simulink model "FCSMPC_double_vector_2025b"  (R2025b)
settings: Solver=FixedStepDiscrete  StartTime=0.0  StopTime=2  FixedStep=SimulinkTs  RelTol=1e-3
PreLoadFcn:
  | % Verzeichnis des Modells zum MATLAB-Pfad hinzufügen
  | modelDir = fileparts(get_param(bdroot, 'FileName'));
  | addpath(modelDir);
  | 
  | % Nur der Dateiname – kein Pfad!
  | set_param(bdroot, 'DataDictionary', 'FOC_params.sldd');
model workspace (MAT data in the model file):
  Np : Simulink.Parameter (value not decoded)
values from neighbouring files (symbols this model uses):
  Filter_Current_FilterTimeConst = 3.3333333333333335E-5    [FOC_params.sldd]
  Filter_Current_SensorTimeConst = 1.5915494309189535E-6    [FOC_params.sldd]
  FOC = evalin("base", "FOC")    [createFOC_SLDD.m]
  FOC_Control_Current_KIid = 10.0    [FOC_params.sldd]
  FOC_Control_Current_KIiq = 10.0    [FOC_params.sldd]
  FOC_Control_Current_KPid = 0.20418507462686566    [FOC_params.sldd]
  FOC_Control_Current_KPiq = 0.58674626865671642    [FOC_params.sldd]
  FOC_Control_Current_Krd = 0.8    [FOC_params.sldd]
  FOC_Control_Current_Krq = 0.8    [FOC_params.sldd]
  FOC_Control_Current_TclCur = 0.1    [FOC_params.sldd]
  FOC_Control_Current_Tnd = 0.1    [FOC_params.sldd]
  FOC_Control_Current_Tnq = 0.1    [FOC_params.sldd]
  FOC_Control_InverterVdc_V = 400.0    [FOC_params.sldd]
  FOC_Control_MotorImax_A = 650.0    [FOC_params.sldd]
  FOC_Control_MTPA_MTPV_nT_id_grid = -450.06704889786266 -439.56177000270145 -427.77784873303676 -416.66404703197372 -406.07553272717422 -395.15516533678584 -384.31176061747851 -374.03652088128132 -363.90551910193739 -353.79478643334204 -344.0221683092833 -334.51243453441936 -324.94614350292119 -315.21793409137081 -305.26543360965195 -295.21828280911944 -285.133916324101 -275.01232812136521 -264.86951532374729 -254.7797625148454 -244    [FOC_params.sldd]
  FOC_Control_MTPA_MTPV_nT_iq_grid = -449.09165648258488 -442.56958748923387 -437.25247759546528 -430.91792082419158 -423.83735797306491 -417.11730433547 -410.54064621830616 -403.71584331167304 -396.93611069310379 -390.15794305727007 -382.97216593027133 -375.44639668848538 -367.93447385667577 -360.57088856352266 -353.41289778449368 -346.34020584402072 -339.28416684923008 -332.22010880540631 -325.11927997033376 -317.92299905654966 -31    [FOC_params.sldd]
  FOC_Control_MTPA_MTPV_T_vec = -245.0 -240.0 -235.0 -230.0 -225.0 -220.0 -215.0 -210.0 -205.0 -200.0 -195.0 -190.0 -185.0 -180.0 -175.0 -170.0 -165.0 -160.0 -155.0 -150.0 -145.0 -140.0 -135.0 -130.0 -125.0 -120.0 -115.0 -110.0 -105.0 -100.0 -95.0 -90.0 -85.0 -80.0 -75.0 -70.0 -65.0 -60.0 -55.0 -50.0 -45.0 -40.0 -35.0 -30.0 -25.0 -20.0 -15.0 -10.0 -5.0 0.0 5.0 10.0 15.0 20.0 25.0 30.0 35.0 40.0 45.0 50.0 55.0 60.0 65.0 70.0 75.0    [FOC_params.sldd]
  FOC_Control_MTPA_MTPV_w_vec = 0.0 10.471975511965978 20.943951023931955 31.415926535897931 41.887902047863911 52.359877559829883 62.831853071795862 73.303828583761828 83.775804095727821 94.247779607693786 104.71975511965977 115.19173063162575 125.66370614359172 136.1356816555577 146.60765716752366 157.07963267948966 167.55160819145564 178.02358370342159 188.49555921538757 198.96753472735358 209.43951023931953 219.9114857512855    [FOC_params.sldd]
  FOC_Control_OpenLoop_Id_Ref_A = 0.0    [FOC_params.sldd]
  FOC_Control_OpenLoop_Iq_Ref_A = 0.0    [FOC_params.sldd]
  FOC_Control_OpenLoop_Ud_OpenLoop_V = 0.0    [FOC_params.sldd]
  FOC_Control_OpenLoop_Uq_OpenLoop_V = 0.0    [FOC_params.sldd]
  FOC_Control_RF_omegamech_rad_s = 3141.5926535897934    [FOC_params.sldd]
  FOC_Control_RF_RateCurrent_A = 500.0    [FOC_params.sldd]
  FOC_Control_RF_RateTrq_Nm = 500.0    [FOC_params.sldd]
  FOC_Control_theta_mechOffsetFix = 0.0    [FOC_params.sldd]
  FOC_Control_theta_mechOffsetTime = 0.0    [FOC_params.sldd]
  FOC_Control_TorqueRef_Nm = 10.0    [FOC_params.sldd]
  FOC_Control_Umax_V = 230.94010767585033    [FOC_params.sldd]
  FOC_Flag_ClosedLoopControl = 1.0    [FOC_params.sldd]
  FOC_Flag_ControlStrategy = 2.0    [FOC_params.sldd]
  FOC_Flag_PWMEnable = 1.0    [FOC_params.sldd]
  FOC_Flag_ResetControl = 0.0    [FOC_params.sldd]
  FOC_Flag_TorqueControl = 1.0    [FOC_params.sldd]
  FOC_LUT_DQLimiter_DQ_LUTScaling = 1.8749999999999995E-5    [FOC_params.sldd]
  FOC_PWM_AZSPWMMethod = 3.0    [FOC_params.sldd]
  FOC_PWM_HybridMode = 1.0    [FOC_params.sldd]
  FOC_PWM_LB1 = 0.5    [FOC_params.sldd]
  FOC_PWM_LB2 = 0.77    [FOC_params.sldd]
  FOC_PWM_PWMManuel = 1.0    [FOC_params.sldd]
  FOC_PWM_RSPWMMethod = 2.0    [FOC_params.sldd]
  FOC_PWM_UB1 = 0.66    [FOC_params.sldd]
  FOC_PWM_UB2 = 0.9    [FOC_params.sldd]
  FOC_SampleTime_TsCur = 0.0001    [FOC_params.sldd]
undefined symbols (not defined in the file or in its folder): dspblkCoreblockFVToolHelper, FCS, Filter, gcbh, Plant, SimulinkTs
libraries: hdlsllib x2, simulink x2, autolibfluxpmsm x1
(part 7 of 8)

== matlab function FCSMPC_double_vector_2025b/FCS_MPC/BuildModel/BuildModel/Discretize_PMSM1 ==
  data: Bd output size=[2 2]; Ld input; Ad output size=[2 2]; Lq input; Rs input; Psi input; wel input; fd output size=[2 1]; Ts input
function [Bd, Ad, fd] = Discretize_PMSM(Ld, Lq, Rs, Psi, wel, Ts)

Ac = [ -Rs/Ld,        wel*Lq/Ld;
    -wel*Ld/Lq,  -Rs/Lq ];

Bc = [ 1/Ld, 0;
    0,    1/Lq ];

fc = [ 0;
    -wel*Psi/Lq ];

% Augmented matrix: states (2) + voltage inputs (2) + affine (1) = 5
M = [ Ac, Bc, fc;
    zeros(3,5) ];

Md = expm(M * Ts);

Ad   = Md(1:2, 1:2);
Bd = Md(1:2, 3:4);     % maps v_dq -> state increment
fd   = Md(1:2, 5);     % back-EMF contribution per step

== matlab function FCSMPC_double_vector_2025b/FCS_MPC/BuildModel/BuildModel/Build_Model1 ==
  data: Ad input; fd input; Gamma output size=[2*Np 2]; Phi output size=[2*Np 1]; Lambdafsw_Ssquare output size=[3*Np 3*Np]; Lambdafsw_SE output size=[3*Np 3]; Apow output size=[2*(Np+1) 2]; Bs_TI output size=[2 3]; Vdc input; lambda_fsw input
function [Gamma, Phi, Lambdafsw_Ssquare, Lambdafsw_SE, Apow, Bs_TI]    = BuildModel(Ad, fd, Vdc, lambda_fsw)
Np = 5;
nu = 3;  ny = 2;
C  = eye(ny);
Apow = zeros(ny*(Np+1), ny);
Apow(1:ny, :) = eye(ny);
for m = 1:Np
    Apow(m*ny + (1:ny), :) = Apow((m-1)*ny + (1:ny), :) * Ad;
end
Bs_TI = switch_to_alphabeta(Vdc);

Gamma = zeros(ny*Np, ny);
Phi   = zeros(ny*Np, 1);
for i = 1:Np
    ri = (i-1)*ny + (1:ny);
    Gamma(ri,:) = C * Apow(i*ny + (1:ny), :);
    acc = zeros(ny,1);
    for m = 0:i-1, acc = acc + Apow(m*ny + (1:ny), :)*fd; end
    Phi(ri) = C * acc;
end

S = eye(nu*Np);
for i = 2:Np
    ri = (i-1)*nu + (1:nu);
    rj = (i-2)*nu + (1:nu);
    S(ri,rj) = -eye(nu);
end
E = [eye(nu); zeros(nu*(Np-1), nu)];
lambda_eff = max(lambda_fsw, 1e-6);
Lambdafsw_SE = lambda_eff * (S.'*E);
Lambdafsw_Ssquare =  lambda_eff*(S.'*S);


end

function Bs_TI = switch_to_alphabeta(Vdc)
Msw = eye(3) - ones(3)/3;
Tc  = (2/3) * [ 1, -1/2,      -1/2;
    0,  sqrt(3)/2, -sqrt(3)/2 ];   % Clarke (2x3)

Bs_TI = Tc * Vdc * Msw;                % 2x3

end

== matlab function FCSMPC_double_vector_2025b/FCS_MPC/SDA_Solve/SDA Solve/QP_Runtime_40k_Simplified_Hybrid ==
  data: H_exp input double size=[15 15]; H_emb input; U_unc_exp output double size=[15 1]; U_unc_emb output; Gamma input double size=[10 2]; Phi input double size=[10 1]; Lambdafsw_SE input double size=[15 3]; Upsil input double size=[10 15]; Bd input double size=[2 2]; Bs_TI input double size=[2 3]; deltaIdqBaseOffset input double size=[2 1]; deltaIdqState input double size=[2 2]; magnitudeGain input double size=[1 1]; phaseCompensation input double size=[2 2]; rippleAttenuation input double size=[1 1]; rippleDelay input double size=[1 1]; Sin_Cos_Theta input double size=[2 1]; idiqFiltered input double size=[2 1]; idiq_ref input double size=[2 1]; lambdaZeroEmbedded input; Ts input double size=[1 1]; U_applied input double size=[6 1]; controllerDelay input double size=[1 1]; iabcPredictedPrevious input double size=[3 1]; Iabc_Motor input double size=[3 1]; predictionValid input boolean size=[1 1]; iabcReconstruction output double size=[3 1]; deltaIabcBase output double size=[3 1]; deltaIabcSwitch output double size=[3 3]; predictionError output double size=[3 1]; reconstructionError output double size=[3 1]; predictionError_dq output double size=[2 1]; reconstructionError_dq output double size=[2 1]; iabcAverageEstimated output double size=[3 1]; iabcRippleEstimated output double size=[3 1]; rippleResidual output double size=[3 1]; iabcSwitchCorrectionRaw output double size=[3 1]
function [U_unc_exp,U_unc_emb,iabcReconstruction, ...
    deltaIabcBase,deltaIabcSwitch, ...
    predictionError,reconstructionError, ...
    predictionError_dq,reconstructionError_dq, ...
    iabcAverageEstimated,iabcRippleEstimated,rippleResidual, ...
    iabcSwitchCorrectionRaw] = ...
    QP_Runtime_40k_Simplified_Hybrid( ...
    H_exp,H_emb,Gamma,Phi,Lambdafsw_SE,Upsil,Bd,Bs_TI, ...
    deltaIdqBaseOffset,deltaIdqState,magnitudeGain,phaseCompensation, ...
    rippleAttenuation,rippleDelay,Sin_Cos_Theta,idiqFiltered, ...
    idiq_ref,lambdaZeroEmbedded,Ts,U_applied,controllerDelay, ...
    iabcPredictedPrevious,Iabc_Motor,predictionValid)
%#codegen
%QP_RUNTIME_40K_SIMPLIFIED_HYBRID Standalone hybrid runtime calculation.
% Current reconstruction is evaluated once. The two matched unconstrained
% centers are then formed using their respective factors and linear terms.

Ts = max(realmin('double'),double(Ts));
idiqFiltered = double(idiqFiltered); idiq_ref = double(idiq_ref);
U_applied = double(U_applied);
lambdaZeroEmbedded = max(0.0,double(lambdaZeroEmbedded));
Bd = double(Bd); Bs_TI = double(Bs_TI);
Sin_Cos_Theta = double(Sin_Cos_Theta);
iabcPredictedPrevious = double(iabcPredictedPrevious);
Iabc_Motor = double(Iabc_Motor);
predictionValid = logical(predictionValid);
uFirst = U_applied(1:3); uSecond = U_applied(4:6);
uAverage = 0.5*(uFirst+uSecond);

sinTheta = Sin_Cos_Theta(1); cosTheta = Sin_Cos_Theta(2);
Rp = [cosTheta, sinTheta; -sinTheta, cosTheta];
TinvClarke = [1.0, 0.0; -0.5, sqrt(3)/2; -0.5, -sqrt(3)/2];
Tclarke = [2/3, -1/3, -1/3; 0, 1/sqrt(3), -1/sqrt(3)];
Tdq2abc = TinvClarke*Rp.'; Tabc2dq = Rp*Tclarke;
deltaIdqSwitch = Bd*Rp*Bs_TI;

deltaIdqBase = deltaIdqState*idiqFiltered+deltaIdqBaseOffset;
period = 2.0*Ts;
rippleAtMeasurementDq = ripple_at_phase( ...
    deltaIdqSwitch,uFirst,uSecond,uAverage,Ts,period-rippleDelay);
rippleResidualDq = ...
    magnitudeGain*rippleAttenuation*rippleAtMeasurementDq;
idiqAverage = phaseCompensation*( ...
    magnitudeGain*idiqFiltered-rippleResidualDq);
idiqAverage = idiqAverage+(rippleDelay/Ts)*( ...
    deltaIdqBase+deltaIdqSwitch*uAverage);
rippleNow = ripple_at_phase( ...
    deltaIdqSwitch,uFirst,uSecond,uAverage,Ts,period);
idiqAtSample = idiqAverage+rippleNow;
delayRatio = min(max(0.0,double(controllerDelay)),Ts)/Ts;
idiqCompensated = idiqAtSample+delayRatio*( ...
    deltaIdqBase+deltaIdqSwitch*uSecond);

iabcReconstruction = Tdq2abc*idiqCompensated;
deltaIabcBase = Tdq2abc*deltaIdqBase;
deltaIabcSwitch = Tdq2abc*deltaIdqSwitch;
iabcAverageEstimated = Tdq2abc*idiqAverage;
iabcRippleEstimated = Tdq2abc*rippleNow;
rippleResidual = Tdq2abc*rippleResidualDq;
iabcAmpCorrected = Tdq2abc*(magnitudeGain*idiqFiltered);
iabcSwitchCorrectionRaw = ...
    (iabcAverageEstimated-iabcAmpCorrected)+iabcRippleEstimated;
if predictionValid
    predictionError = iabcReconstruction-iabcPredictedPrevious;
else
    predictionError = zeros(3,1);
end
reconstructionError = Iabc_Motor-iabcReconstruction;
predictionError_dq = Tabc2dq*predictionError;
reconstructionError_dq = Tabc2dq*reconstructionError;

Np = 5;
r = Gamma*idiqCompensated+Phi-repmat(idiq_ref,Np,1);
F_exp = Upsil.'*r-Lambdafsw_SE*uSecond;
FzeroEmbedded = -0.75*lambdaZeroEmbedded*ones(3*Np,1);
F_emb = F_exp+FzeroEmbedded;
y_exp = H_exp.'\(-F_exp);
U_unc_exp = H_exp\y_exp;
y_emb = H_emb.'\(-F_emb);
U_unc_emb = H_emb\y_emb;
end

function rippleCurrent = ripple_at_phase( ...
    deltaSwitch,uFirst,uSecond,uAverage,vectorStep,t)
period = 2.0*vectorStep;
deltaFirst = deltaSwitch*(uFirst-uAverage);
deltaSecond = deltaSwitch*(uSecond-uAverage);
rippleStart = -0.5*deltaFirst;
t = min(max(0.0,t),period);
if t <= vectorStep
    rippleCurrent = rippleStart+(t/vectorStep)*deltaFirst;
else
    rippleCurrent = rippleStart+deltaFirst+ ...
        ((t-vectorStep)/vectorStep)*deltaSecond;
end
end

== matlab function FCSMPC_double_vector_2025b/FCS_MPC/SDA_Solve/SDA Solve/ SDA_Solve_Synchronized1 ==
  data: H_exp input double size=[15 15]; Jopt output double size=[1 1]; U_unc_exp input double size=[15 1]; H_emb input; U_unc_emb input; NmaxNod input double size=[1 1]; UoptPrev input double size=[15 1]; iabcCompensated input double size=[3 1]; deltaIabcBase input double size=[3 1]; deltaIabcSwitch input double size=[3 3]; lambdaZero input double size=[1 1]; lambdaDeadtime input double size=[1 1]; deadtime_ratio input double size=[1 1]; currentEpsMargin input double size=[1 1]; nodes output double size=[1 1]; optimal output boolean size=[1 1]; Uopt output double size=[15 1]; Uapply output double size=[6 1]; predictionValidNext output boolean size=[1 1]; iabcPredictedNext output double size=[3 1]; leafNodes output double size=[1 1]; bestCMVCost output double size=[1 1]; cmvMetricRatio output double size=[1 1]; switchCountApplied output double size=[1 1]; debug_lower output double size=[3 1]; debug_upper output double size=[3 1]; Jround output double size=[1 1]; Jshift output double size=[1 1]; JbabaiEmbedded output; JbabaiExplicit output; initialRadius output; solutionToggle output boolean size=[1 1]
function [Jopt, nodes, optimal, Uopt, Uapply, ...
    predictionValidNext,iabcPredictedNext, ...
    leafNodes, bestCMVCost, cmvMetricRatio, switchCountApplied, ...
    debug_lower, debug_upper, Jround, Jshift, ...
    JbabaiEmbedded, JbabaiExplicit, initialRadius, solutionToggle] = ...
    SDA_Solve_Synchronized_Hybrid( ...
    H_exp, U_unc_exp, H_emb, U_unc_emb, NmaxNod, UoptPrev, ...
    iabcCompensated, deltaIabcBase, deltaIabcSwitch, ...
    lambdaZero, lambdaDeadtime, deadtime_ratio, currentEpsMargin)
%#codegen
%SDA_SOLVE_SYNCHRONIZED_HYBRID Embedded Babai plus explicit SDA search.
% H_emb/U_unc_emb determine one Babai candidate. That binary sequence is
% re-evaluated under the explicit objective and becomes the initial
% incumbent. Every tree-search center, residual and branch penalty then
% uses H_exp/U_unc_exp. Feed Uopt back through the existing Unit Delay.

Np = 5;
nu = 3;
n = numel(U_unc_exp);

UbarExp = H_exp*U_unc_exp;
UbarEmb = H_emb*U_unc_emb;
uprev = UoptPrev(4:6);
deadtimeRatio = deadtime_ratio;

Uround = min(max(round(U_unc_exp),0.0),1.0);
Ushift = zeros(n,1);
Ushift(1:n-nu) = UoptPrev(nu+1:n);
Ushift(n-nu+1:n) = UoptPrev(n-nu+1:n);

% Forward Babai nearest-plane point for the embedded factor.
% This uses the same conditional centers and binary tie rule as the first
% Schnorr--Euchner descent, but constructs a complete incumbent without
% backtracking.
Ubabai = zeros(n,1);
for babaiLevel = 1:n
    babaiHead = 0.0;
    if babaiLevel > 1
        babaiHead = H_emb(babaiLevel,1:babaiLevel-1)* ...
            Ubabai(1:babaiLevel-1);
    end
    babaiCenter = (UbarEmb(babaiLevel)-babaiHead)/ ...
        H_emb(babaiLevel,babaiLevel);
    if babaiCenter <= 0.5
        Ubabai(babaiLevel) = 0.0;
    else
        Ubabai(babaiLevel) = 1.0;
    end
end

Jround = norm(H_exp*(Uround-U_unc_exp),2)^2;
Jshift = norm(H_exp*(Ushift-U_unc_exp),2)^2;
JbabaiEmbedded = norm(H_emb*(Ubabai-U_unc_emb),2)^2;
JbabaiExplicit = norm(H_exp*(Ubabai-U_unc_exp),2)^2;

% The embedded Babai sequence is the hybrid initializer. Re-evaluating it
% with the explicit factor avoids relying on a hard-coded constant offset.
Uini = Ubabai;
Jini = JbabaiExplicit;

bestCMVCost = sequence_cmv_cost_predicted( ...
    Uini,uprev,iabcCompensated,Np,nu, ...
    deltaIabcBase,deltaIabcSwitch,lambdaZero,lambdaDeadtime, ...
    deadtimeRatio,currentEpsMargin);
bestMetric = Jini+bestCMVCost;
initialRadius = bestMetric;
Uopt = Uini;

U = zeros(n,1);
kidx = ones(n,1);
d2s = zeros(n+1,1);
cmvD2s = zeros(n+1,1);
iabcPrediction = zeros(3,Np+1);
iabcPrediction(:,1) = iabcCompensated;
nodes = 0;
leafNodes = 0;
optimal = true;
i = 1;

while i >= 1
    if kidx(i) > 2
        kidx(i) = 1;
        i = i-1;
        continue;
    end
    head = 0.0;
    if i > 1
        head = H_exp(i,1:i-1)*U(1:i-1);
    end
    center = (UbarExp(i)-head)/H_exp(i,i);
    if center <= 0.5
        firstCandidate = 0.0;
    else
        firstCandidate = 1.0;
    end
    if kidx(i) == 1
        candidate = firstCandidate;
    else
        candidate = 1.0-firstCandidate;
    end
    kidx(i) = kidx(i)+1;
    U(i) = candidate;
    nodes = nodes+1;
    if NmaxNod > 0 && nodes > NmaxNod
        optimal = false;
        break;
    end

    residual = UbarExp(i)-head-H_exp(i,i)*candidate;
    metricNew = d2s(i)+residual*residual;
    cmvMetricNew = cmvD2s(i);
    if mod(i,nu) == 0
        predictionStep = i/nu;
        blockStart = i-nu+1;
        uCurrent = U(blockStart:i);
        if predictionStep == 1
            uPrevious = uprev;
        else
            uPrevious = U(blockStart-nu:blockStart-1);
        end
        iabcBeforeSwitch = iabcPrediction(:,predictionStep);
        [deltaStep,deltaDead] = deadtime_corrected_current_step( ...
            uPrevious,uCurrent,iabcBeforeSwitch, ...
            deltaIabcBase,deltaIabcSwitch,deadtimeRatio,currentEpsMargin);
        cmvIncrement = cmv_cost( ...
            uPrevious,uCurrent,iabcBeforeSwitch,deltaDead, ...
            lambdaZero,lambdaDeadtime,currentEpsMargin);
        metricNew = metricNew+cmvIncrement;
        cmvMetricNew = cmvMetricNew+cmvIncrement;
        iabcPrediction(:,predictionStep+1) = iabcBeforeSwitch+deltaStep;
    end
    if metricNew > bestMetric
        continue;
    end
    if i == n
        leafNodes = leafNodes+1;
        if metricNew < bestMetric
            bestMetric = metricNew;
            Uopt = U;
            bestCMVCost = cmvMetricNew;
        end
    else
        d2s(i+1) = metricNew;
        cmvD2s(i+1) = cmvMetricNew;
        i = i+1;
        kidx(i) = 1;
    end
end

if ~isfinite(bestMetric)
    Uopt = repmat(uprev,Np,1);
end

Uapply = Uopt(1:6);
UapplyFirst = Uopt(1:3);
UapplySecond = Uopt(4:6);

[deltaFirst,~] = deadtime_corrected_current_step( ...
    uprev,UapplyFirst,iabcCompensated, ...
    deltaIabcBase,deltaIabcSwitch, ...
    deadtimeRatio,currentEpsMargin);
iabcAfterFirst = iabcCompensated + deltaFirst;

[deltaSecond,~] = deadtime_corrected_current_step( ...
    UapplyFirst,UapplySecond,iabcAfterFirst, ...
    deltaIabcBase,deltaIabcSwitch,deadtimeRatio,currentEpsMargin);
iabcPredictedNext = iabcAfterFirst+deltaSecond;

switchCountApplied = sum(abs(UapplyFirst-uprev))+ ...
    sum(abs(UapplySecond-UapplyFirst));
Jopt = bestMetric;
if Jopt > eps
    cmvMetricRatio = bestCMVCost/Jopt;
else
    cmvMetricRatio = 0.0;
end
[~,debugDeltaDead] = deadtime_corrected_current_step( ...
    uprev,UapplyFirst,iabcCompensated,deltaIabcBase,deltaIabcSwitch, ...
    deadtimeRatio,currentEpsMargin);
[~,debug_lower,debug_upper] = cmv_cost( ...
    uprev,UapplyFirst,iabcCompensated,debugDeltaDead, ...
    lambdaZero,lambdaDeadtime,currentEpsMargin);
predictionValidNext = true;

% Toggle once after every completed SDA solution. The downstream switch
% detects this edge and explicitly restarts from the first vector.
persistent solutionToggleState
if isempty(solutionToggleState)
    solutionToggleState = false;
end
solutionToggleState = ~solutionToggleState;
solutionToggle = solutionToggleState;
end

function [deltaStep,deltaDead] = deadtime_corrected_current_step( ...
    uPrevious,uCurrent,iabcBeforeSwitch, ...
    deltaBase,deltaSwitch,deadtimeRatio,currentEps)
uDead = uCurrent;
changed = (uPrevious ~= uCurrent);
signEps = 0.1*currentEps;
for phase = 1:3
    if ~changed(phase)
        continue;
    end
    iPhase = iabcBeforeSwitch(phase);
    if iPhase >= signEps
        uDead(phase) = 0.0;
    elseif iPhase <= -signEps
        uDead(phase) = 1.0;
    else
        uDead(phase) = 0.5*(1.0-iPhase/signEps);
    end
end
uEffective = deadtimeRatio*uDead+(1.0-deadtimeRatio)*uCurrent;
deltaDead = deadtimeRatio*(deltaBase+deltaSwitch*uDead);
deltaStep = deltaBase+deltaSwitch*uEffective;
end

function [penalty,lowerBound,upperBound] = cmv_cost( ...
    uPrevious,uCurrent,iabcBeforeSwitch,deltaDead, ...
    lambdaZero,lambdaDeadtime,currentEpsMargin)
penalty = 0.0;
iabcDeadEnd = iabcBeforeSwitch+deltaDead;
lowerBound = min(iabcBeforeSwitch,iabcDeadEnd)-currentEpsMargin;
upperBound = max(iabcBeforeSwitch,iabcDeadEnd)+currentEpsMargin;
uncertain = (lowerBound <= 0.0) & (upperBound >= 0.0);
if all(uCurrent == 0.0) || all(uCurrent == 1.0)
    penalty = penalty+lambdaZero;
end
changed = (uPrevious ~= uCurrent);
if sum(changed) ~= 2
    return;
end
canBeZero = false(3,1);
canBeOne = false(3,1);
for phase = 1:3
    if ~changed(phase)
        canBeZero(phase) = (uPrevious(phase) == 0.0);
        canBeOne(phase) = (uPrevious(phase) == 1.0);
    elseif uncertain(phase)
        canBeZero(phase) = true;
        canBeOne(phase) = true;
    elseif iabcDeadEnd(phase) > 0.0
        canBeZero(phase) = true;
    else
        canBeOne(phase) = true;
    end
end
if all(canBeZero) || all(canBeOne)
    penalty = penalty+lambdaDeadtime;
end
end

function totalPenalty = sequence_cmv_cost_predicted( ...
    U,uprev,iabcInitial,Np,nu,deltaBase,deltaSwitch, ...
    lambdaZero,lambdaDeadtime,deadtimeRatio,currentEpsMargin)
totalPenalty = 0.0;
uPrevious = uprev;
iabcBeforeSwitch = iabcInitial;
for step = 1:Np
    rows = (step-1)*nu+(1:nu);
    uCurrent = U(rows);
    [deltaStep,deltaDead] = deadtime_corrected_current_step( ...
        uPrevious,uCurrent,iabcBeforeSwitch,deltaBase,deltaSwitch, ...
        deadtimeRatio,currentEpsMargin);
    totalPenalty = totalPenalty+cmv_cost( ...
        uPrevious,uCurrent,iabcBeforeSwitch,deltaDead, ...
        lambdaZero,lambdaDeadtime,currentEpsMargin);
    iabcBeforeSwitch = iabcBeforeSwitch+deltaStep;
    uPrevious = uCurrent;
end
end

== stateflow chart FCSMPC_double_vector_2025b/FCS_MPC/CurrentRefCalc/Current_RateLimiter/RateLimiter ==
  settings: updateMethod=DISCRETE  sampleTime=FOC.SampleTime.TsSpeed
  state IDLE
  state Rising
    entry:  y =  fi(y_prev +dT * R, 1, 32, 18);
    exit: y_prev = y;
  state Falling
    entry:  y = fi(y_prev+dT * F, 1, 32, 18);
    exit: y_prev = y;
  state Directpassage
    entry:  y = u;
    exit: y_prev = y;
  (default) -> IDLE
  IDLE -> (junction 22)
  (junction 22) -> Rising [order 1] : [(u-y_prev)/dT>=R]
  (junction 22) -> Falling [order 2] : [(u-y_prev)/dT<=F]
  Rising -> (junction 22)
  Falling -> (junction 22)
  Directpassage -> (junction 22)
  (junction 22) -> Directpassage [order 3] : [(u-y_prev)/dT<R && (u-y_prev)/dT>F]
  data: u input fixdt(1,32,18); R input fixdt(1,32,18); F input fixdt(1,32,18); dT constant fixdt(1,32,18) size=1 =FOC.SampleTime.TsSpeed; y output fixdt(1,32,18); y_prev local fixdt(1,32,18) =0

== matlab function FCSMPC_double_vector_2025b/FCS_MPC/SDA_Solve/SDA Solve/ SDA_Solve_Synchronized2 ==
  data: H_exp input double size=[15 15]; Jopt output double size=[1 1]; U_unc_exp input double size=[15 1]; H_emb input; U_unc_emb input; NmaxNod input double size=[1 1]; UoptPrev input double size=[15 1]; iabcCompensated input double size=[3 1]; deltaIabcBase input double size=[3 1]; deltaIabcSwitch input double size=[3 3]; lambdaZero input double size=[1 1]; lambdaDeadtime input double size=[1 1]; deadtime_ratio input double size=[1 1]; currentEpsMargin input double size=[1 1]; nodes output double size=[1 1]; optimal output boolean size=[1 1]; Uopt output double size=[15 1]; Uapply output double size=[6 1]; predictionValidNext output boolean size=[1 1]; iabcPredictedNext output double size=[3 1]; leafNodes output double size=[1 1]; bestCMVCost output double size=[1 1]; cmvMetricRatio output double size=[1 1]; switchCountApplied output double size=[1 1]; debug_lower output double size=[3 1]; debug_upper output double size=[3 1]; Jround output double size=[1 1]; Jshift output double size=[1 1]; JbabaiEmbedded output; JbabaiExplicit output; initialRadius output; solutionToggle output boolean size=[1 1]; currentLimit input; feasibleSolutionFound output; babaiPrefixFeasible output; prefixRepairUsed output; feasiblePrefixCount output; currentPruneCount output
function [Jopt, nodes, optimal, Uopt, Uapply, ...
    predictionValidNext,iabcPredictedNext, ...
    leafNodes, bestCMVCost, cmvMetricRatio, switchCountApplied, ...
    debug_lower, debug_upper, Jround, Jshift, ...
    JbabaiEmbedded, JbabaiExplicit, initialRadius, solutionToggle, ...
    feasibleSolutionFound, babaiPrefixFeasible, prefixRepairUsed, ...
    feasiblePrefixCount, currentPruneCount] = ...
    SDA_Solve_Synchronized_Hybrid_CurrentConstrained( ...
    H_exp, U_unc_exp, H_emb, U_unc_emb, NmaxNod, UoptPrev, ...
    iabcCompensated, deltaIabcBase, deltaIabcSwitch, ...
    lambdaZero, lambdaDeadtime, deadtime_ratio, currentEpsMargin, ...
    currentLimit)
%#codegen
%SDA_SOLVE_SYNCHRONIZED_HYBRID_CURRENTCONSTRAINED
% Current-constrained extension of SDA_Solve_Synchronized_Hybrid.
%
% The ordinary embedded Babai sequence remains the fast path. Its first two
% switching blocks, which are applied before the next controller transaction,
% are checked at both the dead-time endpoint and the vector endpoint. If that
% prefix is infeasible, all feasible two-block prefixes are scored only by the
% six-level embedded partial metric. The best prefix is completed once with a
% conditional embedded Babai suffix and reevaluated with the full explicit
% objective. The explicit search retains every feasible prefix and performs
% current pruning after each of the first two complete switching blocks.
%
% currentLimit is a phase-current peak limit in amperes. A nonpositive or
% nonfinite value disables the current constraint for diagnostic use.

Np = 5;
nu = 3;
n = numel(U_unc_exp);
constrainedBlocks = 2;

UbarExp = H_exp*U_unc_exp;
UbarEmb = H_emb*U_unc_emb;
uprev = UoptPrev(4:6);
deadtimeRatio = deadtime_ratio;
constraintEnabled = isfinite(currentLimit) && currentLimit > 0.0;

Uround = min(max(round(U_unc_exp),0.0),1.0);
Ushift = zeros(n,1);
Ushift(1:n-nu) = UoptPrev(nu+1:n);
Ushift(n-nu+1:n) = UoptPrev(n-nu+1:n);

% Ordinary embedded Babai candidate.
Ubabai = zeros(n,1);
for babaiLevel = 1:n
    babaiHead = 0.0;
    if babaiLevel > 1
        babaiHead = H_emb(babaiLevel,1:babaiLevel-1)* ...
            Ubabai(1:babaiLevel-1);
    end
    babaiCenter = (UbarEmb(babaiLevel)-babaiHead)/ ...
        H_emb(babaiLevel,babaiLevel);
    Ubabai(babaiLevel) = double(babaiCenter > 0.5);
end

Jround = norm(H_exp*(Uround-U_unc_exp),2)^2;
Jshift = norm(H_exp*(Ushift-U_unc_exp),2)^2;
JbabaiEmbedded = norm(H_emb*(Ubabai-U_unc_emb),2)^2;
JbabaiExplicit = norm(H_exp*(Ubabai-U_unc_exp),2)^2;

[babaiCMVCost,babaiPrefixFeasible] = evaluate_sequence( ...
    Ubabai,uprev,iabcCompensated,Np,nu, ...
    deltaIabcBase,deltaIabcSwitch,lambdaZero,lambdaDeadtime, ...
    deadtimeRatio,currentEpsMargin,currentLimit, ...
    constrainedBlocks,constraintEnabled);

prefixRepairUsed = false;
feasiblePrefixCount = 0;
hasFeasibleIncumbent = false;
Uini = zeros(n,1);
Jini = inf;
bestCMVCost = 0.0;

if babaiPrefixFeasible
    % Preserve the existing hybrid fast path exactly when it is feasible.
    Uini = Ubabai;
    Jini = JbabaiExplicit;
    bestCMVCost = babaiCMVCost;
    hasFeasibleIncumbent = true;
else
    prefixRepairUsed = true;
    bestPrefixMetric = inf;
    bestPrefix = zeros(2*nu,1);

    % Enumerate only the physical two-vector prefix. No Babai suffix is
    % formed inside this loop. The selected prefix is the feasible point
    % nearest to the unconstrained center in the first six embedded rows.
    for state1 = 0:7
        u1 = state_from_index(state1);
        [delta1,deltaDead1] = deadtime_corrected_current_step( ...
            uprev,u1,iabcCompensated,deltaIabcBase,deltaIabcSwitch, ...
            deadtimeRatio,currentEpsMargin);
        iDead1 = iabcCompensated+deltaDead1;
        iAfter1 = iabcCompensated+delta1;
        if ~current_is_feasible(iDead1,iAfter1,currentLimit, ...
                constraintEnabled)
            continue;
        end

        for state2 = 0:7
            u2 = state_from_index(state2);
            [delta2,deltaDead2] = deadtime_corrected_current_step( ...
                u1,u2,iAfter1,deltaIabcBase,deltaIabcSwitch, ...
                deadtimeRatio,currentEpsMargin);
            iDead2 = iAfter1+deltaDead2;
            iAfter2 = iAfter1+delta2;
            if ~current_is_feasible(iDead2,iAfter2,currentLimit, ...
                    constraintEnabled)
                continue;
            end

            feasiblePrefixCount = feasiblePrefixCount+1;
            prefix = [u1;u2];
            prefixResidual = UbarEmb(1:2*nu)- ...
                H_emb(1:2*nu,1:2*nu)*prefix;
            prefixMetric = prefixResidual.'*prefixResidual;
            if prefixMetric < bestPrefixMetric
                bestPrefixMetric = prefixMetric;
                bestPrefix = prefix;
            end
        end
    end

    if feasiblePrefixCount > 0
        % Compute exactly one conditional embedded Babai suffix.
        Uini(1:2*nu) = bestPrefix;
        for babaiLevel = 2*nu+1:n
            babaiHead = H_emb(babaiLevel,1:babaiLevel-1)* ...
                Uini(1:babaiLevel-1);
            babaiCenter = (UbarEmb(babaiLevel)-babaiHead)/ ...
                H_emb(babaiLevel,babaiLevel);
            Uini(babaiLevel) = double(babaiCenter > 0.5);
        end

        Jini = norm(H_exp*(Uini-U_unc_exp),2)^2;
        [bestCMVCost,initialCandidateFeasible] = evaluate_sequence( ...
            Uini,uprev,iabcCompensated,Np,nu, ...
            deltaIabcBase,deltaIabcSwitch,lambdaZero,lambdaDeadtime, ...
            deadtimeRatio,currentEpsMargin,currentLimit, ...
            constrainedBlocks,constraintEnabled);
        hasFeasibleIncumbent = initialCandidateFeasible;
    end
end

if hasFeasibleIncumbent
    bestMetric = Jini+bestCMVCost;
    Uopt = Uini;
else
    % An infeasible candidate may guide ordering but is never a finite upper
    % bound. The first feasible leaf found by the main search establishes it.
    bestMetric = inf;
    initialRadius = inf;
    Uopt = zeros(n,1);
    bestCMVCost = 0.0;
end
if hasFeasibleIncumbent
    initialRadius = bestMetric;
end

U = zeros(n,1);
kidx = ones(n,1);
d2s = zeros(n+1,1);
cmvD2s = zeros(n+1,1);
iabcPrediction = zeros(3,Np+1);
iabcPrediction(:,1) = iabcCompensated;
nodes = 0;
leafNodes = 0;
currentPruneCount = 0;
optimal = true;
i = 1;

while i >= 1
    if kidx(i) > 2
        kidx(i) = 1;
        i = i-1;
        continue;
    end
    head = 0.0;
    if i > 1
        head = H_exp(i,1:i-1)*U(1:i-1);
    end
    center = (UbarExp(i)-head)/H_exp(i,i);
    firstCandidate = double(center > 0.5);
    if kidx(i) == 1
        candidate = firstCandidate;
    else
        candidate = 1.0-firstCandidate;
    end
    kidx(i) = kidx(i)+1;
    U(i) = candidate;
    nodes = nodes+1;
    if NmaxNod > 0 && nodes > NmaxNod
        optimal = false;
        break;
    end

    residual = UbarExp(i)-head-H_exp(i,i)*candidate;
    metricNew = d2s(i)+residual*residual;
    cmvMetricNew = cmvD2s(i);
    currentFeasible = true;
    if mod(i,nu) == 0
        predictionStep = i/nu;
        blockStart = i-nu+1;
        uCurrent = U(blockStart:i);
        if predictionStep == 1
            uPrevious = uprev;
        else
            uPrevious = U(blockStart-nu:blockStart-1);
        end
        iabcBeforeSwitch = iabcPrediction(:,predictionStep);
        [deltaStep,deltaDead] = deadtime_corrected_current_step( ...
            uPrevious,uCurrent,iabcBeforeSwitch, ...
            deltaIabcBase,deltaIabcSwitch,deadtimeRatio,currentEpsMargin);
        iabcDeadEnd = iabcBeforeSwitch+deltaDead;
        iabcAfterStep = iabcBeforeSwitch+deltaStep;

        if predictionStep <= constrainedBlocks
            currentFeasible = current_is_feasible( ...
                iabcDeadEnd,iabcAfterStep,currentLimit,constraintEnabled);
        end
        if ~currentFeasible
            currentPruneCount = currentPruneCount+1;
            continue;
        end

        cmvIncrement = cmv_cost( ...
            uPrevious,uCurrent,iabcBeforeSwitch,deltaDead, ...
            lambdaZero,lambdaDeadtime,currentEpsMargin);
        metricNew = metricNew+cmvIncrement;
        cmvMetricNew = cmvMetricNew+cmvIncrement;
        iabcPrediction(:,predictionStep+1) = iabcAfterStep;
    end

    if hasFeasibleIncumbent && metricNew > bestMetric
        continue;
    end
    if i == n
        leafNodes = leafNodes+1;
        if ~hasFeasibleIncumbent || metricNew < bestMetric
            bestMetric = metricNew;
            Uopt = U;
            bestCMVCost = cmvMetricNew;
            hasFeasibleIncumbent = true;
        end
    else
        d2s(i+1) = metricNew;
        cmvD2s(i+1) = cmvMetricNew;
        i = i+1;
        kidx(i) = 1;
    end
end

feasibleSolutionFound = hasFeasibleIncumbent;
if ~feasibleSolutionFound
    % Keep the output deterministic but mark it invalid explicitly. The caller
    % must provide a separately validated safety fallback for this condition.
    Uopt = repmat(uprev,Np,1);
    bestMetric = inf;
    bestCMVCost = 0.0;
end

Uapply = Uopt(1:6);
UapplyFirst = Uopt(1:3);
UapplySecond = Uopt(4:6);

[deltaFirst,~] = deadtime_corrected_current_step( ...
    uprev,UapplyFirst,iabcCompensated, ...
    deltaIabcBase,deltaIabcSwitch,deadtimeRatio,currentEpsMargin);
iabcAfterFirst = iabcCompensated+deltaFirst;
[deltaSecond,~] = deadtime_corrected_current_step( ...
    UapplyFirst,UapplySecond,iabcAfterFirst, ...
    deltaIabcBase,deltaIabcSwitch,deadtimeRatio,currentEpsMargin);
iabcPredictedNext = iabcAfterFirst+deltaSecond;

switchCountApplied = sum(abs(UapplyFirst-uprev))+ ...
    sum(abs(UapplySecond-UapplyFirst));
Jopt = bestMetric;
if isfinite(Jopt) && Jopt > eps
    cmvMetricRatio = bestCMVCost/Jopt;
else
    cmvMetricRatio = 0.0;
end
[~,debugDeltaDead] = deadtime_corrected_current_step( ...
    uprev,UapplyFirst,iabcCompensated,deltaIabcBase,deltaIabcSwitch, ...
    deadtimeRatio,currentEpsMargin);
[~,debug_lower,debug_upper] = cmv_cost( ...
    uprev,UapplyFirst,iabcCompensated,debugDeltaDead, ...
    lambdaZero,lambdaDeadtime,currentEpsMargin);
predictionValidNext = feasibleSolutionFound;

persistent solutionToggleState
if isempty(solutionToggleState)
    solutionToggleState = false;
end
solutionToggleState = ~solutionToggleState;
solutionToggle = solutionToggleState;
end

function u = state_from_index(stateIndex)
u = zeros(3,1);
u(1) = floor(stateIndex/4);
u(2) = floor(mod(stateIndex,4)/2);
u(3) = mod(stateIndex,2);
end

function feasible = current_is_feasible( ...
    iabcDeadEnd,iabcAfterStep,currentLimit,constraintEnabled)
if ~constraintEnabled
    feasible = true;
else
    feasible = all(abs(iabcDeadEnd) <= currentLimit) && ...
        all(abs(iabcAfterStep) <= currentLimit);
end
end

function [deltaStep,deltaDead] = deadtime_corrected_current_step( ...
    uPrevious,uCurrent,iabcBeforeSwitch, ...
    deltaBase,deltaSwitch,deadtimeRatio,currentEps)
uDead = uCurrent;
changed = (uPrevious ~= uCurrent);
signEps = 0.1*currentEps;
for phase = 1:3
    if ~changed(phase)
        continue;
    end
    iPhase = iabcBeforeSwitch(phase);
    if iPhase >= signEps
        uDead(phase) = 0.0;
    elseif iPhase <= -signEps
        uDead(phase) = 1.0;
    else
        uDead(phase) = 0.5*(1.0-iPhase/signEps);
    end
end
uEffective = deadtimeRatio*uDead+(1.0-deadtimeRatio)*uCurrent;
deltaDead = deadtimeRatio*(deltaBase+deltaSwitch*uDead);
deltaStep = deltaBase+deltaSwitch*uEffective;
end

function [penalty,lowerBound,upperBound] = cmv_cost( ...
    uPrevious,uCurrent,iabcBeforeSwitch,deltaDead, ...
    lambdaZero,lambdaDeadtime,currentEpsMargin)
penalty = 0.0;
iabcDeadEnd = iabcBeforeSwitch+deltaDead;
lowerBound = min(iabcBeforeSwitch,iabcDeadEnd)-currentEpsMargin;
upperBound = max(iabcBeforeSwitch,iabcDeadEnd)+currentEpsMargin;
uncertain = (lowerBound <= 0.0) & (upperBound >= 0.0);
if all(uCurrent == 0.0) || all(uCurrent == 1.0)
    penalty = penalty+lambdaZero;
end
changed = (uPrevious ~= uCurrent);
if sum(changed) ~= 2
    return;
end
canBeZero = false(3,1);
canBeOne = false(3,1);
for phase = 1:3
    if ~changed(phase)
        canBeZero(phase) = (uPrevious(phase) == 0.0);
        canBeOne(phase) = (uPrevious(phase) == 1.0);
    elseif uncertain(phase)
        canBeZero(phase) = true;
        canBeOne(phase) = true;
    elseif iabcDeadEnd(phase) > 0.0
        canBeZero(phase) = true;
    else
        canBeOne(phase) = true;
    end
end
if all(canBeZero) || all(canBeOne)
    penalty = penalty+lambdaDeadtime;
end
end

function [totalPenalty,prefixFeasible] = evaluate_sequence( ...
    U,uprev,iabcInitial,Np,nu,deltaBase,deltaSwitch, ...
    lambdaZero,lambdaDeadtime,deadtimeRatio,currentEpsMargin, ...
    currentLimit,constrainedBlocks,constraintEnabled)
totalPenalty = 0.0;
prefixFeasible = true;
uPrevious = uprev;
iabcBeforeSwitch = iabcInitial;
for step = 1:Np
    rows = (step-1)*nu+(1:nu);
    uCurrent = U(rows);
    [deltaStep,deltaDead] = deadtime_corrected_current_step( ...
        uPrevious,uCurrent,iabcBeforeSwitch,deltaBase,deltaSwitch, ...
        deadtimeRatio,currentEpsMargin);
    iabcDeadEnd = iabcBeforeSwitch+deltaDead;
    iabcAfterStep = iabcBeforeSwitch+deltaStep;
    if step <= constrainedBlocks && ...
            ~current_is_feasible(iabcDeadEnd,iabcAfterStep, ...
            currentLimit,constraintEnabled)
        prefixFeasible = false;
        return;
    end
    totalPenalty = totalPenalty+cmv_cost( ...
        uPrevious,uCurrent,iabcBeforeSwitch,deltaDead, ...
        lambdaZero,lambdaDeadtime,currentEpsMargin);
    iabcBeforeSwitch = iabcAfterStep;
    uPrevious = uCurrent;
end
end
